simulink model "EV_drive_cycle"  (R2025a)
settings: Solver=VariableStepAuto  StartTime=0.0  StopTime=765  RelTol=1e-3
settings Model: Creator=Shashwat Sinha  LastModifiedBy=navan

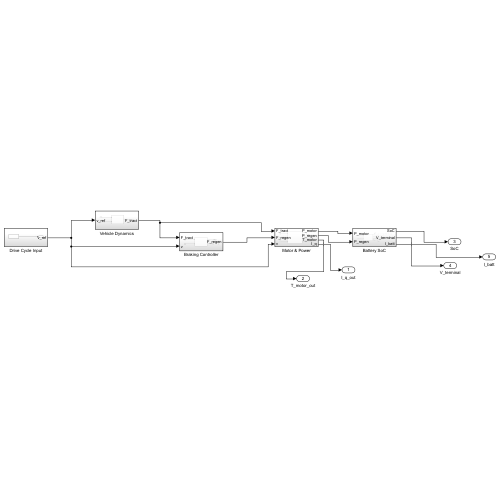
[thumbnail: Simulink's stored preview of the top-level diagram]
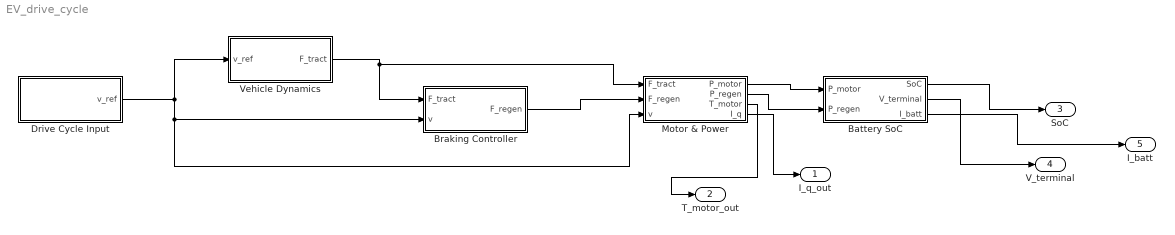
== system EV_drive_cycle ==
  Battery SoC : Subsystem
  Braking Controller : Subsystem
  Drive Cycle Input : Subsystem
  Motor & Power : Subsystem
  Vehicle Dynamics : Subsystem
  I_q_out : Outport
  T_motor_out : Outport  Port=2
  SoC : Outport  Port=3
  V_terminal : Outport  Port=4
  I_batt : Outport  Port=5
  wires:
  Drive Cycle Input/1(v_ref) -> Motor & Power/3(v), Braking Controller/2(v), Vehicle Dynamics/1(v_ref)
  Vehicle Dynamics/1(F_tract) -> Motor & Power/1(F_tract), Braking Controller/1(F_tract)
  Braking Controller/1(F_regen) -> Motor & Power/2(F_regen)
  Motor & Power/1(P_motor) -> Battery SoC/1(P_motor)
  Motor & Power/2(P_regen) -> Battery SoC/2(P_regen)
  Motor & Power/4(I_q) -> I_q_out/1
  Motor & Power/3(T_motor) -> T_motor_out/1
  Battery SoC/1(SoC) -> SoC/1
  Battery SoC/2(V_terminal) -> V_terminal/1
  Battery SoC/3(I_batt) -> I_batt/1

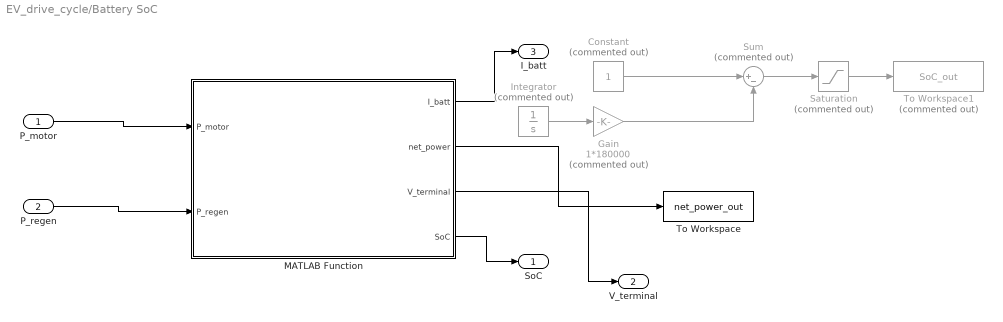
== system EV_drive_cycle/Battery SoC ==
  P_motor : Inport
  P_regen : Inport  Port=2
  Constant : Constant  Commented=on
  Gain : Gain  Commented=on  Gain=1*180000
  Integrator : Integrator  Commented=on
  MATLAB Function : MATLAB Function  TreatAsAtomicUnit=on
  Saturation : Saturate  Commented=on  UpperLimit=1  LowerLimit=0
  Sum : Sum  Commented=on  Inputs=|+-
  To Workspace : ToWorkspace  VariableName=net_power_out  SaveFormat=Timeseries  SampleTime=-1
  To Workspace1 : ToWorkspace  Commented=on  VariableName=SoC_out  SaveFormat=Timeseries  SampleTime=-1
  SoC : Outport
  V_terminal : Outport  Port=2
  I_batt : Outport  Port=3
  wires:
  MATLAB Function/1(I_batt) -> I_batt/1
  P_motor/1 -> MATLAB Function/1(P_motor)
  P_regen/1 -> MATLAB Function/2(P_regen)
  Integrator/1 -> Gain/1
  Gain/1 -> Sum/2
  Constant/1 -> Sum/1
  Sum/1 -> Saturation/1
  Saturation/1 -> To Workspace1/1
  MATLAB Function/2(net_power) -> To Workspace/1
  MATLAB Function/4(SoC) -> SoC/1
  MATLAB Function/3(V_terminal) -> V_terminal/1

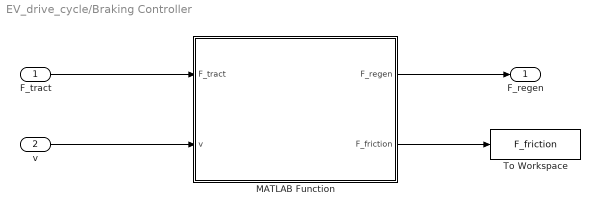
== system EV_drive_cycle/Braking Controller ==
  F_tract : Inport
  v : Inport  Port=2
  MATLAB Function : MATLAB Function  TreatAsAtomicUnit=on
  To Workspace : ToWorkspace  VariableName=F_friction  SaveFormat=Timeseries  SampleTime=-1
  F_regen : Outport
  wires:
  F_tract/1 -> MATLAB Function/1(F_tract)
  v/1 -> MATLAB Function/2(v)
  MATLAB Function/2(F_friction) -> To Workspace/1
  MATLAB Function/1(F_regen) -> F_regen/1

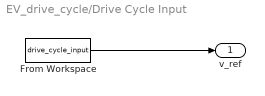
== system EV_drive_cycle/Drive Cycle Input ==
  From Workspace : FromWorkspace  VariableName=drive_cycle_input  SampleTime=0.1
  v_ref : Outport
  wires:
  From Workspace/1 -> v_ref/1

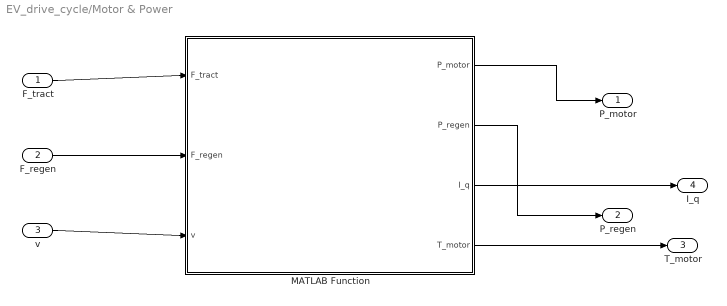
== system EV_drive_cycle/Motor & Power ==
  F_tract : Inport
  F_regen : Inport  Port=2
  v : Inport  Port=3
  MATLAB Function : MATLAB Function  TreatAsAtomicUnit=on
  P_motor : Outport
  P_regen : Outport  Port=2
  T_motor : Outport  Port=3
  I_q : Outport  Port=4
  wires:
  F_tract/1 -> MATLAB Function/1(F_tract)
  F_regen/1 -> MATLAB Function/2(F_regen)
  v/1 -> MATLAB Function/3(v)
  MATLAB Function/1(P_motor) -> P_motor/1
  MATLAB Function/2(P_regen) -> P_regen/1
  MATLAB Function/4(T_motor) -> T_motor/1
  MATLAB Function/3(I_q) -> I_q/1

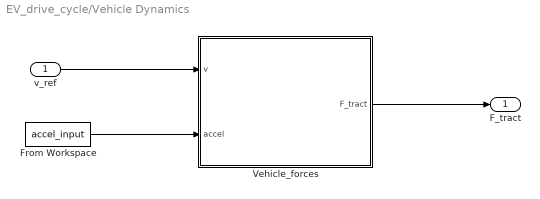
== system EV_drive_cycle/Vehicle Dynamics ==
  v_ref : Inport
  From Workspace : FromWorkspace  VariableName=accel_input  SampleTime=0.1
  Vehicle_forces : MATLAB Function  TreatAsAtomicUnit=on
  F_tract : Outport
  wires:
  From Workspace/1 -> Vehicle_forces/2(accel)
  v_ref/1 -> Vehicle_forces/1(v)
  Vehicle_forces/1(F_tract) -> F_tract/1

== matlab function EV_drive_cycle/Braking Controller/MATLAB Function ==
  data: F_tract input; F_regen output; v input; F_friction output
function [F_regen, F_friction] = braking_controller(F_tract, v)
    if F_tract >= 0
        % Accelerating — no braking
        F_regen = 0;
        F_friction = 0;
    elseif v > 15
        % Full regen
        F_regen = F_tract;
        F_friction = 0;
    elseif v > 5
        % Partial regen (linear blend)
        regen_ratio = (v - 5) / 10;
        F_regen = F_tract * regen_ratio;
        F_friction = F_tract * (1 - regen_ratio);
    else
        % Low speed — friction only
        F_regen = 0;
        F_friction = F_tract;
    end
end

== matlab function EV_drive_cycle/Vehicle Dynamics/Vehicle_forces ==
  data: v input; F_tract output; accel input
function F_tract = vehicle_dynamics(v, accel)
    % Vehicle parameters
    m = 1500;       % kg
    Cd = 0.28;
    A = 2.2;        % m^2
    rho = 1.225;    % kg/m^3
    Crr = 0.01;
    g = 9.81;

    F_aero = 0.5 * rho * Cd * A * v^2;
    F_roll = m * g * Crr;
    F_inertia = m * accel;

    F_tract = F_inertia + F_aero + F_roll;
end

== matlab function EV_drive_cycle/Motor & Power/MATLAB Function ==
  data: F_tract input; P_motor output; F_regen input; v input; P_regen output; I_q output; T_motor output
function [P_motor, P_regen, I_q, T_motor] = motor_power_fcn(F_tract, F_regen, v)
%#codegen
% Replaces the flat 92%/85% efficiency model with:
%   - electrical current lag (armature/winding inductance)
%   - torque-speed limiting from a real motor curve
%   - copper (I^2R) + iron (speed^2) losses
%   - lumped thermal model with torque derating when hot

persistent I_q_state T_motor_state initialized
if isempty(initialized)
    I_q_state = 0;
    T_motor_state = 25;      % degC, ambient start
    initialized = true;
end

%% Fixed parameters
dt        = 0.1;     % s, must match model sample time
r_wheel   = 0.30;     % m
G         = 9.0;      % gear ratio (wheel <- motor)
Kt        = 1.2;      % Nm/A, torque constant
R_phase   = 0.05;     % ohm, winding resistance
tau_elec  = 0.05;      % s, electrical time constant (L/R lag)
k_iron    = 2e-5;      % iron loss coefficient (W per (rad/s)^2)
Nbase_rpm = 5000; Nmax_rpm = 17000;
Tcont     = 181.5;      % Nm (95kW / Nbase from your torque.m)
Tpeak     = 375;        % Nm
C_th      = 4000;       % J/degC, thermal mass of motor+housing
h_cool    = 25;         % W/degC, cooling to ambient
T_amb     = 25;         % degC
T_derate_start = 120;   % degC, torque starts derating
T_max     = 150;        % degC, hard cutoff

%% Kinematics
omega_motor = (v / r_wheel) * G;              % rad/s
rpm         = omega_motor * 60/(2*pi);

%% Torque request from vehicle-dynamics force
T_req = (F_tract - F_regen) * r_wheel / G;    % Nm at motor shaft

%% Speed-dependent torque limit (peak envelope, matches torque.m)
if abs(rpm) <= Nbase_rpm
    T_limit = Tpeak;
else
    Ppeak_kW = Tpeak * (Nbase_rpm*pi/30) * 1e-3;
    T_limit  = (Ppeak_kW*1e3) / max(abs(omega_motor), 1e-3);
end

%% Thermal derating
if T_motor_state > T_max
    derate = 0;
elseif T_motor_state > T_derate_start
    derate = (T_max - T_motor_state) / (T_max - T_derate_start);
else
    derate = 1;
end
T_limit = T_limit * derate;
T_cmd   = max(min(T_req, T_limit), -T_limit);

%% Electrical current dynamics (1st order lag toward commanded current)
I_cmd = T_cmd / Kt;
I_q_state = I_q_state + (dt/tau_elec) * (I_cmd - I_q_state);
T_actual  = Kt * I_q_state;

%% Losses
P_copper = I_q_state^2 * R_phase;             % W
P_iron   = k_iron * omega_motor^2;            % W
P_mech   = T_actual * omega_motor;            % W (signed)

%% Split into motoring / regen electrical power (bus side)
if P_mech >= 0
    P_motor = P_mech + P_copper + P_iron;     % drawing from battery
    P_regen = 0;
else
    regen_eff = 0.85;
    P_regen = -P_mech * regen_eff - P_copper - P_iron;
    P_regen = max(P_regen, 0);
    P_motor = 0;
end

%% Thermal update
P_loss = P_copper + P_iron;
T_motor_state = T_motor_state + (dt/C_th) * (P_loss - h_cool*(T_motor_state - T_amb));

I_q     = I_q_state;
T_motor = T_motor_state;

== matlab function EV_drive_cycle/Battery SoC/MATLAB Function ==
  data: P_motor input; I_batt output; P_regen input; net_power output; V_terminal output; SoC output
function [I_batt, net_power, V_terminal, SoC] = battery_soc_fcn(P_motor, P_regen)
%#codegen
% Replaces fixed-360V Coulomb counting with a 1st-order Thevenin
% equivalent circuit: Voc(SoC) lookup + series resistance R0 + one RC pair.
% This gives real terminal-voltage sag under load and a transient response,
% instead of SoC being a pure linear ramp.

persistent SoC_state Vc1_state I_prev initialized
if isempty(initialized)
    SoC_state = 1.0;     % start full
    Vc1_state = 0;
    I_prev    = 0;
    initialized = true;
end

%% Fixed parameters
dt      = 0.1;         % s
Q_batt  = 50 * 3600;    % 50 Ah -> Coulombs
R0      = 0.05;          % ohm, internal series resistance
R1      = 0.03;          % ohm, RC branch resistance
C1      = 2000;          % F, RC branch capacitance (~60s transient)

% Simple OCV(SoC) curve for a 360V nominal Li-ion pack (typical shape)
SoC_bp  = [0    0.1   0.2   0.4   0.6   0.8   0.9   1.0];
Voc_bp  = [320  345   355   362   367   372   378   392];  % V

net_power = P_motor - P_regen;   % W, positive = drawing from battery

%% Open circuit voltage at current SoC
Voc = interp1(SoC_bp, Voc_bp, SoC_state, 'linear', 'extrap');

%% Solve for battery current from P = V_t * I, V_t = Voc - I*R0 - Vc1
% Quadratic: -R0*I^2 + (Voc - Vc1_state)*I - net_power = 0
a = -R0;
b = (Voc - Vc1_state);
c = -net_power;
disc = b^2 - 4*a*c;
if disc < 0
    disc = 0;   % numeric guard
end
I1 = (-b + sqrt(disc)) / (2*a);
I2 = (-b - sqrt(disc)) / (2*a);
% Pick the physically sensible root (smaller magnitude current)
if abs(I1) <= abs(I2)
    I_batt = I1;
else
    I_batt = I2;
end

%% RC branch dynamics
Vc1_state = Vc1_state + (dt/C1) * (I_batt - Vc1_state/R1);

%% Terminal voltage
V_terminal = Voc - I_batt*R0 - Vc1_state;

%% Coulomb counting for SoC (now on top of the dynamic current, not a flat one)
SoC_state = SoC_state - (I_batt * dt) / Q_batt;
SoC_state = max(min(SoC_state, 1), 0);

I_prev = I_batt;
SoC    = SoC_state;
